simulink model "etapa02_buck_simscape"  (R2026a)
settings: Solver=ode23t  MaxStep=1e-6  RelTol=1e-4
values from neighbouring files (symbols this model uses):
  Ts = 1e-4    (= 0.0001)    [circuito_completo_parametros.m]    (also in etapa01_referencia.m; etapa02_projeto_buck.m; etapa02_simulink.m; etapa03_projeto_ccs.m)
undefined symbols (not defined in the file or in its folder): Rload
libraries: fl_lib x9, nesl_utility x4, simulink x1
settings Model: Creator=pedro  LastModifiedBy=pedro

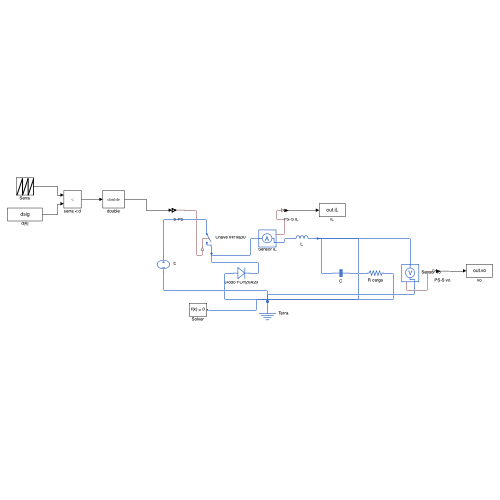
[thumbnail: Simulink's stored preview of the top-level diagram]
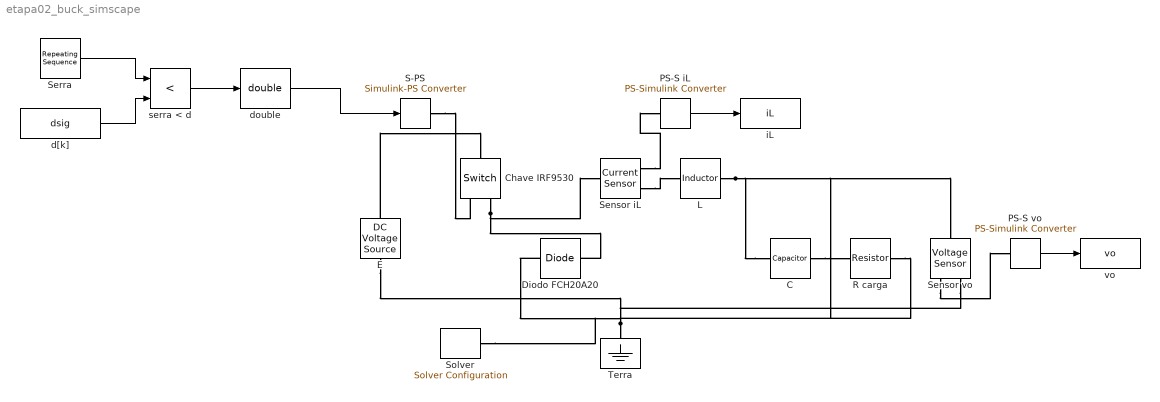
== system etapa02_buck_simscape ==
  C : fl_lib/Electrical/Electrical Elements/Capacitor  c=Cval F  r=0 Ohm  g=0 1/Ohm  i_specify=off  i_priority=None  i=0 A  i_nominal_specify=off  i_nominal_value=1  i_nominal_unit=A  v_specify=off  v_priority=None  v=0 V  v_nominal_specify=off  v_nominal_value=1  v_nominal_unit=V  vc_specify=off  vc_priority=High  vc=0 V  vc_nominal_specify=off  vc_nominal_value=1  vc_nominal_unit=V
  Chave IRF9530 : fl_lib/Electrical/Electrical Elements/Switch  R_closed=Ron Ohm  G_open=1e-9 1/Ohm  Threshold=0.5  i_specify=off  i_priority=None  i=0 A  i_nominal_specify=off  i_nominal_value=1  i_nominal_unit=A  v_specify=off  v_priority=None  v=0 V  v_nominal_specify=off  v_nominal_value=1  v_nominal_unit=V
  Diodo FCH20A20 : fl_lib/Electrical/Electrical Elements/Diode  Vf=Vf V  Ron=Rd Ohm  Goff=1e-9 1/Ohm  i_specify=off  i_priority=None  i=0 A  i_nominal_specify=off  i_nominal_value=1  i_nominal_unit=A  v_specify=off  v_priority=None  v=0 V  v_nominal_specify=off  v_nominal_value=1  v_nominal_unit=V
  E : fl_lib/Electrical/Electrical Sources/DC Voltage Source  v0=E V
  L : fl_lib/Electrical/Electrical Elements/Inductor  l=Lval H  r=RL Ohm  g=0 1/Ohm  i_specify=off  i_priority=None  i=0 A  i_nominal_specify=off  i_nominal_value=1  i_nominal_unit=A  v_specify=off  v_priority=None  v=0 V  v_nominal_specify=off  v_nominal_value=1  v_nominal_unit=V  i_L_specify=off  i_L_priority=High  i_L=0 A  i_L_nominal_specify=off  i_L_nominal_value=1  i_L_nominal_unit=A
  PS-S iL : nesl_utility/PS-Simulink Converter  PhysicalDomain=network_engine_domain  SubClassName=ps_output  LeftPortType=input  RightPortType=output  PseudoPeriodic=off  Frequencies=[]  VectorFormat=inherit  Unit=A  AffineConversion=off
  PS-S vo : nesl_utility/PS-Simulink Converter  PhysicalDomain=network_engine_domain  SubClassName=ps_output  LeftPortType=input  RightPortType=output  PseudoPeriodic=off  Frequencies=[]  VectorFormat=inherit  Unit=V  AffineConversion=off
  R carga : fl_lib/Electrical/Electrical Elements/Resistor  R=Rload Ohm  i_specify=off  i_priority=None  i=0 A  i_nominal_specify=off  i_nominal_value=1  i_nominal_unit=A  v_specify=off  v_priority=None  v=0 V  v_nominal_specify=off  v_nominal_value=1  v_nominal_unit=V
  S-PS : nesl_utility/Simulink-PS Converter  PhysicalDomain=network_engine_domain  SubClassName=ps_input  LeftPortType=input  RightPortType=output  PseudoPeriodic=off  Frequencies=[]  NoiseDistribution=none  NoiseParameters=[]  Unit=1  AffineConversion=off  FilteringAndDerivatives=zero  SimscapeFilterOrder=1  InputFilterTimeConstant=0.001  UdotUserProvided=0
  Sensor iL : fl_lib/Electrical/Electrical Sensors/Current Sensor
  Sensor vo : fl_lib/Electrical/Electrical Sensors/Voltage Sensor
  Serra : simulink/Sources/Repeating Sequence  rep_seq_t=[0 Ts]  rep_seq_y=[0 1]
  Solver : nesl_utility/Solver Configuration  PhysicalDomain=network_engine_domain  SubClassName=solver  LeftPortType=input  RightPortType=generic  Tones=[]  Harmonics=[]  SimulateNoise=off  Profile=off  UseLocalSampling=off  EnableSwitchedLinearOptims=on  FrequencyDomain=off  UseCCode=off  RelTol=0.001  AbsTol=0.001  MinStep=1e-09  ToWorkspace=off  RevertToSquareIcSolve=off  NumHomotopyIterations=100  PhasorMode=off  PhasorModeNumHarmonics=1  ConsistencySolver=NEWTON_XTOL_AFTER_FTOL  CanonicalOrdering=CANONICAL  OptimizeIntermediates=OPTIMIZED  IndexReductionMethod=DerivativeReplacement  DoDC=off  ResidualTolerance=1e-09  ConsistencyTolSource=GLOBAL  ConsistencyAbsTol=0.001  ConsistencyRelTol=0.001  ConsistencyTolFactor=0.001  UseLocalSolver=off  LocalSolverChoice=NE_BACKWARD_EULER_ADVANCER  ResolveIndetEquations=on  FunctionEvalNumThread=1  LocalSolverSampleTime=0.001  DoFixedCost=off  MaxNonlinIter=3  MaxModeIter=2  ComputeImpulses=off  ImpulseIterations=2  LinearAlgebra=auto  LinearAlgebraNumThread=0  EquationFormulation=NE_TIME_EF  DelaysMemoryBudget=1024  AutomaticFiltering=on  FilteringTimeConstant=0.001  PartitionStorageMethod=AS_NEEDED  PartitionMemoryBudget=1024  PartitionMethod=ROBUST  MultibodyUseLocalSolver=off  MultibodyLocalSolverChoice=ODE1  MultibodyLocalSolverSampleTime=0.001
  Terra : fl_lib/Electrical/Electrical Elements/Electrical Reference
  d[k] : FromWorkspace  VariableName=dsig  Interpolate=off  OutputAfterFinalValue=Holding final value
  double : DataTypeConversion  OutDataTypeStr=double  SaturateOnIntegerOverflow=off  RndMeth=Floor
  iL : ToWorkspace  VariableName=iL  SaveFormat=Timeseries  SampleTime=-1
  serra < d : RelationalOperator  Operator=<  OutDataTypeStr=boolean  RndMeth=Simplest  InputSameDT=off
  vo : ToWorkspace  VariableName=vo  SaveFormat=Timeseries  SampleTime=-1
  wires:
  Serra/1 -> serra < d/1
  d[k]/1 -> serra < d/2
  serra < d/1 -> double/1
  double/1 -> S-PS/1
  PS-S iL/1 -> iL/1
  PS-S vo/1 -> vo/1
  connections:
  E/LConn1 -- Chave IRF9530/LConn1
  Diodo FCH20A20/RConn1 -- Chave IRF9530/RConn2 -- Sensor iL/LConn1
  Sensor iL/RConn2 -- L/LConn1
  C/LConn1 -- L/RConn1 -- R carga/LConn1 -- Sensor vo/LConn1
  E/RConn1 -- Diodo FCH20A20/LConn1 -- C/RConn1 -- R carga/RConn1 -- Sensor vo/RConn2 -- Terra/LConn1 -- Solver/RConn1
  S-PS/RConn1 -- Chave IRF9530/RConn1
  Sensor iL/RConn1 -- PS-S iL/LConn1
  Sensor vo/RConn1 -- PS-S vo/LConn1
